simulink model "easybike_battery"  (R2024a)
settings: Solver=VariableStepAuto  StartTime=0.0  StopTime=10.0  RelTol=1e-3
PreLoadFcn:
  | easybike_init;
values from neighbouring files (symbols this model uses):
  Ah_nom = P_.Ah(1)    [easybike_init.m]
  CFtab = interp1(P_.Tbp, P_.CF(1,:), Tbp)    [easybike_init.m]
  OCVtab = [P_.V(1) P_.V(1)]    [easybike_init.m]
  Pw = P.ekm*P.speed    [easybike_build_simulink.m]    (also in easybike_discharge.m; easybike_init.m = P_.ekm*P_.speed)
  R25 = (1-eta0)*eta0*V^2/Pw    [easybike_discharge.m]    (also in easybike_init.m = (1-sqrt(P_.RTE(1)))*sqrt(P_.RTE(1))*P_.V(1)^2/Pw)
  RFtab = exp(P_.Er(1)*1000/8.314*(1./(Tbp+273.15) - 1/298.15))    [easybike_init.m]
  SOCbp = [0 1]    [easybike_init.m]
  Tbp = [0 5 10 15 20 25 30 35 40 45 50]    [easybike_init.m]
  Tcell_C = 30    [easybike_init.m]
settings Model: Creator=Razowan  LastModifiedBy=Razowan

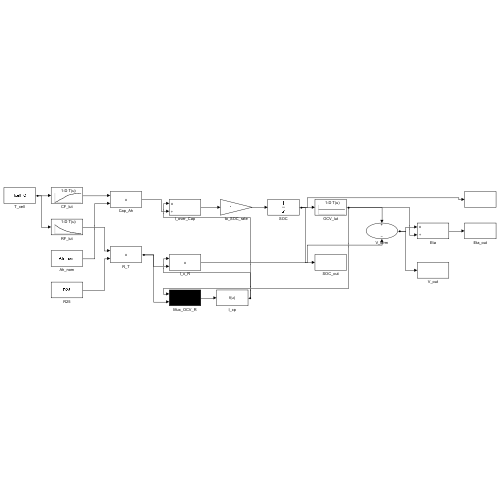
[thumbnail: Simulink's stored preview of the top-level diagram]
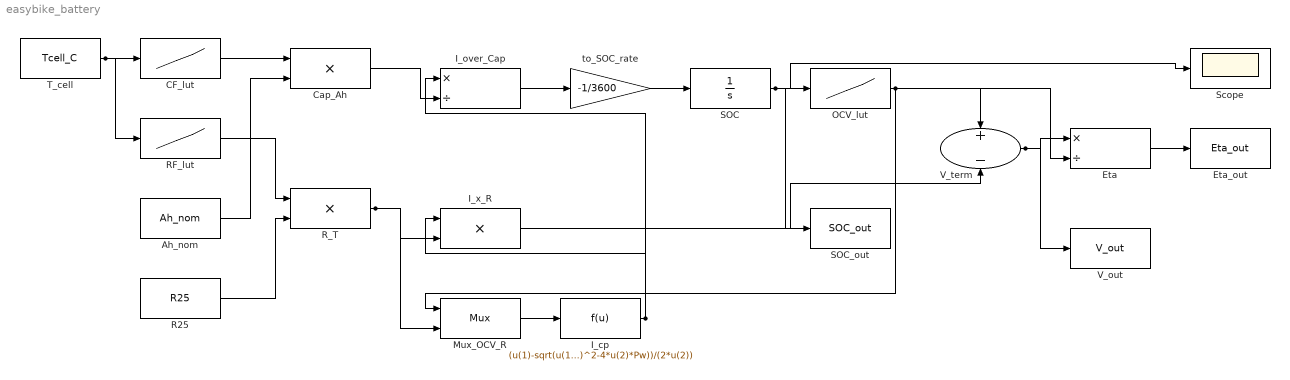
== system easybike_battery ==
  Ah_nom : Constant  Value=Ah_nom
  CF_lut : Lookup_n-D  NumberOfTableDimensions=1  BreakpointsForDimension1=Tbp  Table=CFtab  InternalRulePriority=Speed  RndMeth=Simplest
  Cap_Ah : Product  Inputs=**
  Eta : Product  Inputs=*/
  Eta_out : ToWorkspace  VariableName=Eta_out  SampleTime=-1
  I_cp : Fcn  Expr=(u(1)-sqrt(u(1)^2-4*u(2)*Pw))/(2*u(2))
  I_over_Cap : Product  Inputs=*/
  I_x_R : Product  Inputs=**
  Mux_OCV_R : Mux  Inputs=2
  OCV_lut : Lookup_n-D  NumberOfTableDimensions=1  BreakpointsForDimension1=SOCbp  Table=OCVtab  InternalRulePriority=Speed  RndMeth=Simplest
  R25 : Constant  Value=R25
  RF_lut : Lookup_n-D  NumberOfTableDimensions=1  BreakpointsForDimension1=Tbp  Table=RFtab  InternalRulePriority=Speed  RndMeth=Simplest
  R_T : Product  Inputs=**
  SOC : Integrator  InitialCondition=1  LimitOutput=on  UpperSaturationLimit=1  LowerSaturationLimit=0
  SOC_out : ToWorkspace  VariableName=SOC_out  SampleTime=-1
  Scope : Scope
  T_cell : Constant  Value=Tcell_C
  V_out : ToWorkspace  VariableName=V_out  SampleTime=-1
  V_term : Sum  Inputs=+-
  to_SOC_rate : Gain  Gain=-1/3600
  wires:
  T_cell/1 -> CF_lut/1, RF_lut/1
  CF_lut/1 -> Cap_Ah/1
  Ah_nom/1 -> Cap_Ah/2
  RF_lut/1 -> R_T/1
  R25/1 -> R_T/2
  OCV_lut/1 -> Mux_OCV_R/1, V_term/1, Eta/2
  R_T/1 -> Mux_OCV_R/2, I_x_R/2
  Mux_OCV_R/1 -> I_cp/1
  I_cp/1 -> I_over_Cap/1, I_x_R/1
  Cap_Ah/1 -> I_over_Cap/2
  I_over_Cap/1 -> to_SOC_rate/1
  to_SOC_rate/1 -> SOC/1
  SOC/1 -> OCV_lut/1, SOC_out/1, Scope/1
  I_x_R/1 -> V_term/2
  V_term/1 -> Eta/1, V_out/1
  Eta/1 -> Eta_out/1
